simulink model "sm_car_"  (R2026b)
settings: Solver=ode23t  StopTime=100  MaxStep=0.4  AbsTol=1e-3  EnableMultiTasking=on
PreLoadFcn:
  | % Due to usability issue in Repeating Sequence block
  | warning('off','Simulink:Masking:Invalid');
  | 
  | % Eliminate unnecessary warnings in inactive variants
  | % Warnings generated only if you click through inactive variant
  | warning('off','MATLAB:nonExistentField');
  | warning('off','Simulink:Parameters:BlkParamUndefined');
PostLoadFcn:
  | set_param([bdroot '/Vehicle'],'popup_trailer','Off')
  | warning('off','sm:sli:setup:compile:LocalSolverNotSupported')
  | %sm_car_config_maneuver(bdroot,'WOT Braking');
  | sm_car_config_vehicle(bdroot,'false');
  | sm_car_config_logging(bdroot);
InitFcn:
  | sm_car_config_camera;
  | Vehicle = sm_car_vehcfg_checkConfig(Vehicle);
  | sm_car_check_tire_model(bdroot);
StartFcn:
  | tic;
StopFcn:
  | Elapsed_Sim_Time = toc;
  | % disp(['Elapsed Sim Time = ' num2str(Elapsed_Sim_Time)]);
undefined symbols (not defined in the file or in its folder): acc_theta, accel_ramp_rate, Axle1D, AxleIn, Camera, Control, Driver, Init, Maneuver, Pedal, Scene, ShaftL1, ShaftL2, ShaftR1, ShaftR2, Visual, X, xy_data_car_side, Y, Z
libraries: sm_lib x290, fl_lib x171, nesl_utility x144, simulink x60, simulink_extras x14, sdl_lib x14, SimscapeFluids_lib x7, Damper_Element x4, Tire_1x2x x4, ee_lib x3, Scene_Utilities x3, sharedTrackingLibrary x2
(part 8 of 22)

== system sm_car_/Vehicle/Vehicle/Powertrain ==
  CtrlD : Inport
  CtrlP : Inport  Port=2
  VehB : Inport  Port=3
  Driveline : Subsystem  Tag=PublishSubsystem  Variant=on  VariantControlMode=label  VariantControl=Shaft  LabelModeActiveChoice=L2_R2  mask(Variants for Driveline){Driveline=Powertrain.Driveline, VariantLabel=Powertrain.Driveline.class.Value}
      mask prompts: Driveline "Driveline Parameters"; VariantLabel "Variant Label"
      mask help: Select option and provide parameters for driveline. Option is chosen by string provided in Variant Label. The parameters for the selected option are contained in Driveline data structure.
      mask init:
      | curblk = gcb;
      | 
      | % Set variant for this block 
      | set_param(curblk,'LabelModeActiveChoice',VariantLabel);
      settings: AttributesFormatString=%<ActiveVariant>
      mask Help: web('sm_car_doc_driveline.html');
  Power : Subsystem  Variant=on  VariantControlMode=label  VariantControl=Variant1  LabelModeActiveChoice=Electric_L2_R2  mask(Variants for Power){Power=Powertrain.Power, VariantLabel=Powertrain.Power.class.Value}
      mask prompts: Power "Power Parameters"; VariantLabel "Variant Label"
      mask help: Select option and provide parameters for power system (energy storage and actuator). Option is chosen by string provided in Variant Label. The parameters for the selected option are contained in Power data structure.
      mask init:
      | curblk = gcb;
      | 
      | % Set variant for this block 
      | set_param(curblk,'LabelModeActiveChoice',VariantLabel);
      settings: AttributesFormatString=%<ActiveVariant>
  FA : PMIOPort  Side=Left
  Ref : PMIOPort  Port=2  Side=Right
  RA : PMIOPort  Port=3  Side=Right
  R1 : PMIOPort  Port=4  Side=Right
  L1 : PMIOPort  Port=5  Side=Left
  L2 : PMIOPort  Port=6  Side=Left
  R2 : PMIOPort  Port=7  Side=Right
  OutD : Outport  VectorParamsAs1DForOutWhenUnconnected=off
  OutP : Outport  Port=2  VectorParamsAs1DForOutWhenUnconnected=off
  wires:
  Driveline/1(OutD) -> OutD/1
  CtrlD/1 -> Driveline/1(CtrlBus)
  Power/1(OutP) -> OutP/1
  CtrlP/1 -> Power/1(CtrlBus)
  VehB/1 -> Power/2(VehBus)
  connections:
  Driveline/LConn1 -- FA/RConn1
  Ref/RConn1 -- Power/RConn1
  Driveline/RConn1 -- RA/RConn1
  Driveline/LConn4 -- Power/LConn1
  Driveline/LConn2 -- L1/RConn1
  Driveline/RConn2 -- R1/RConn1
  Driveline/RConn3 -- R2/RConn1
  Driveline/LConn3 -- L2/RConn1

== system sm_car_/Vehicle/Vehicle Constraint/No Constraint ==
  F : PMIOPort  Side=Right
  B : PMIOPort  Port=2  Side=Left

== system sm_car_/Vehicle/Vehicle Constraint/No Yaw ==
  Cartesian Joint : sm_lib/Joints/Cartesian Joint  JointMode=Normal  CompositeWrenchDir=FollowerOnBase  CompositeWrenchFrame=BaseFrame  SenseConstraintForce=off  SenseConstraintTorque=off  SenseTotalForce=off  SenseTotalTorque=off  PxPositionTargetSpecify=off  PxPositionTargetPriority=High  PxPositionTargetValue=0  PxPositionTargetValueUnits=m  PxVelocityTargetSpecify=off  PxVelocityTargetPriority=High  PxVelocityTargetValue=0  PxVelocityTargetValueUnits=m/s  PxEquilibriumPosition=0  PxEquilibriumPositionUnits=m  PxSpringStiffness=0  PxSpringStiffnessUnits=N/m  PxDampingCoefficient=0  PxDampingCoefficientUnits=N/(m/s)  PxLowerLimitSpecify=off  PxLowerLimitBound=-1  PxLowerLimitBoundUnits=m  PxLowerLimitStiffness=1e6  PxLowerLimitStiffnessUnits=N/m  PxLowerLimitDamping=1e3  PxLowerLimitDampingUnits=N/(m/s)  PxLowerLimitTransitionRegionWidth=1e-4  PxLowerLimitTransitionRegionWidthUnits=m  PxUpperLimitSpecify=off  PxUpperLimitBound=1  PxUpperLimitBoundUnits=m  PxUpperLimitStiffness=1e6  PxUpperLimitStiffnessUnits=N/m  PxUpperLimitDamping=1e3  PxUpperLimitDampingUnits=N/(m/s)  PxUpperLimitTransitionRegionWidth=1e-4  PxUpperLimitTransitionRegionWidthUnits=m  PxTorqueActuationMode=NoTorque  PxMotionActuationMode=ComputedMotion  PxSensePosition=off  PxSenseVelocity=off  PxSenseAcceleration=off  PxSenseTorqueForce=off  PxSenseLowerLimitTorqueForce=off  PxSenseUpperLimitTorqueForce=off  PyPositionTargetSpecify=off  PyPositionTargetPriority=High  PyPositionTargetValue=0  PyPositionTargetValueUnits=m  PyVelocityTargetSpecify=off  PyVelocityTargetPriority=High  PyVelocityTargetValue=0  PyVelocityTargetValueUnits=m/s  PyEquilibriumPosition=0  PyEquilibriumPositionUnits=m  PySpringStiffness=0  PySpringStiffnessUnits=N/m  PyDampingCoefficient=0  PyDampingCoefficientUnits=N/(m/s)  PyLowerLimitSpecify=off  PyLowerLimitBound=-1  PyLowerLimitBoundUnits=m  PyLowerLimitStiffness=1e6  PyLowerLimitStiffnessUnits=N/m  PyLowerLimitDamping=1e3  PyLowerLimitDampingUnits=N/(m/s)  PyLowerLimitTransitionRegionWidth=1e-4  PyLowerLimitTransitionRegionWidthUnits=m  PyUpperLimitSpecify=off  PyUpperLimitBound=1  PyUpperLimitBoundUnits=m  PyUpperLimitStiffness=1e6  PyUpperLimitStiffnessUnits=N/m  PyUpperLimitDamping=1e3  PyUpperLimitDampingUnits=N/(m/s)  PyUpperLimitTransitionRegionWidth=1e-4  PyUpperLimitTransitionRegionWidthUnits=m  PyTorqueActuationMode=NoTorque  PyMotionActuationMode=ComputedMotion  PySensePosition=off  PySenseVelocity=off  PySenseAcceleration=off  PySenseTorqueForce=off  PySenseLowerLimitTorqueForce=off  PySenseUpperLimitTorqueForce=off  PzPositionTargetSpecify=off  PzPositionTargetPriority=High  PzPositionTargetValue=0  PzPositionTargetValueUnits=m  PzVelocityTargetSpecify=off  PzVelocityTargetPriority=High  PzVelocityTargetValue=0  PzVelocityTargetValueUnits=m/s  PzEquilibriumPosition=0  PzEquilibriumPositionUnits=m  PzSpringStiffness=0  PzSpringStiffnessUnits=N/m  PzDampingCoefficient=0  PzDampingCoefficientUnits=N/(m/s)  PzLowerLimitSpecify=off  PzLowerLimitBound=-1  PzLowerLimitBoundUnits=m  PzLowerLimitStiffness=1e6  PzLowerLimitStiffnessUnits=N/m  PzLowerLimitDamping=1e3  PzLowerLimitDampingUnits=N/(m/s)  PzLowerLimitTransitionRegionWidth=1e-4  PzLowerLimitTransitionRegionWidthUnits=m  PzUpperLimitSpecify=off  PzUpperLimitBound=1  PzUpperLimitBoundUnits=m  PzUpperLimitStiffness=1e6  PzUpperLimitStiffnessUnits=N/m  PzUpperLimitDamping=1e3  PzUpperLimitDampingUnits=N/(m/s)  PzUpperLimitTransitionRegionWidth=1e-4  PzUpperLimitTransitionRegionWidthUnits=m  PzTorqueActuationMode=NoTorque  PzMotionActuationMode=ComputedMotion  PzSensePosition=off  PzSenseVelocity=off  PzSenseAcceleration=off  PzSenseTorqueForce=off  PzSenseLowerLimitTorqueForce=off  PzSenseUpperLimitTorqueForce=off
  Universal Joint : sm_lib/Joints/Universal Joint  JointMode=Normal  CompositeWrenchDir=FollowerOnBase  CompositeWrenchFrame=BaseFrame  SenseConstraintForce=off  SenseConstraintTorque=off  SenseTotalForce=off  SenseTotalTorque=off  RxPositionTargetSpecify=off  RxPositionTargetPriority=High  RxPositionTargetValue=0  RxPositionTargetValueUnits=deg  RxVelocityTargetSpecify=off  RxVelocityTargetPriority=High  RxVelocityTargetValue=0  RxVelocityTargetValueUnits=deg/s  RxEquilibriumPosition=0  RxEquilibriumPositionUnits=deg  RxSpringStiffness=0  RxSpringStiffnessUnits=N*m/deg  RxDampingCoefficient=0  RxDampingCoefficientUnits=N*m/(deg/s)  RxLowerLimitSpecify=off  RxLowerLimitBound=-90  RxLowerLimitBoundUnits=deg  RxLowerLimitStiffness=1e4  RxLowerLimitStiffnessUnits=N*m/deg  RxLowerLimitDamping=10  RxLowerLimitDampingUnits=N*m/(deg/s)  RxLowerLimitTransitionRegionWidth=0.1  RxLowerLimitTransitionRegionWidthUnits=deg  RxUpperLimitSpecify=off  RxUpperLimitBound=90  RxUpperLimitBoundUnits=deg  RxUpperLimitStiffness=1e4  RxUpperLimitStiffnessUnits=N*m/deg  RxUpperLimitDamping=10  RxUpperLimitDampingUnits=N*m/(deg/s)  RxUpperLimitTransitionRegionWidth=0.1  RxUpperLimitTransitionRegionWidthUnits=deg  RxTorqueActuationMode=NoTorque  RxMotionActuationMode=ComputedMotion  RxSensePosition=off  RxSenseVelocity=off  RxSenseAcceleration=off  RxSenseTorqueForce=off  RxSenseLowerLimitTorqueForce=off  RxSenseUpperLimitTorqueForce=off  RyPositionTargetSpecify=off  RyPositionTargetPriority=High  RyPositionTargetValue=0  RyPositionTargetValueUnits=deg  RyVelocityTargetSpecify=off  RyVelocityTargetPriority=High  RyVelocityTargetValue=0  RyVelocityTargetValueUnits=deg/s  RyEquilibriumPosition=0  RyEquilibriumPositionUnits=deg  RySpringStiffness=0  RySpringStiffnessUnits=N*m/deg  RyDampingCoefficient=0  RyDampingCoefficientUnits=N*m/(deg/s)  RyLowerLimitSpecify=off  RyLowerLimitBound=-90  RyLowerLimitBoundUnits=deg  RyLowerLimitStiffness=1e4  RyLowerLimitStiffnessUnits=N*m/deg  RyLowerLimitDamping=10  RyLowerLimitDampingUnits=N*m/(deg/s)  RyLowerLimitTransitionRegionWidth=0.1  RyLowerLimitTransitionRegionWidthUnits=deg  RyUpperLimitSpecify=off  RyUpperLimitBound=90  RyUpperLimitBoundUnits=deg  RyUpperLimitStiffness=1e4  RyUpperLimitStiffnessUnits=N*m/deg  RyUpperLimitDamping=10  RyUpperLimitDampingUnits=N*m/(deg/s)  RyUpperLimitTransitionRegionWidth=0.1  RyUpperLimitTransitionRegionWidthUnits=deg  RyTorqueActuationMode=NoTorque  RyMotionActuationMode=ComputedMotion  RySensePosition=off  RySenseVelocity=off  RySenseAcceleration=off  RySenseTorqueForce=off  RySenseLowerLimitTorqueForce=off  RySenseUpperLimitTorqueForce=off
  F : PMIOPort  Side=Right
  B : PMIOPort  Port=2  Side=Left
  connections:
  Cartesian Joint/LConn1 -- B/RConn1
  Cartesian Joint/RConn1 -- Universal Joint/LConn1
  Universal Joint/RConn1 -- F/RConn1

== system sm_car_/Visualization/Unreal/Animation Off ==
  xyz : Inport
  rpy : Inport  Port=2
  ws : Inport  Port=3
  aCamber : Inport  Port=4
  aSteerWheel : Inport  Port=5
  Terminator{,1..4} (5 alike) : Terminator
  wires:
  rpy/1 -> Terminator1/1
  aSteerWheel/1 -> Terminator4/1
  aCamber/1 -> Terminator3/1
  xyz/1 -> Terminator/1
  ws/1 -> Terminator2/1

== system sm_car_/World/Mechanism Configuration/Constant Gravity ==
  MechanismConfiguration : sm_lib/Utilities/Mechanism Configuration  UniformGravity=Constant  GravityVector=GravityVector  GravityVectorUnits=m/s^2  LinearizationDelta=0.001  JointModeTransitionNonlinearIterations=2
  C : PMIOPort  Side=Right
  connections:
  MechanismConfiguration/RConn1 -- C/RConn1

== system sm_car_/World/Mechanism Configuration/Variable GravityXY ==
  Constant : Constant  Value=acc_theta
  Constant1 : Constant  Value=GravityVector(3)
  MechanismConfiguration : sm_lib/Utilities/Mechanism Configuration  UniformGravity=TimeVarying  GravityVector=[0 0 -9.80665]  GravityVectorUnits=m/s^2  LinearizationDelta=0.001  JointModeTransitionNonlinearIterations=2
  Mux : Mux  Inputs=3
  Product : Product
  Product1 : Product
  Ramp1 : simulink/Sources/Ramp  slope=accel_ramp_rate  start=2  InitialOutput=0
  Scope : Scope
      settings: ActiveDisplayYMinimum=-1.12718  ActiveDisplayYMaximum=10.14459
  Simulink-PS Converter : nesl_utility/Simulink-PS Converter  PhysicalDomain=network_engine_domain  SubClassName=ps_input  LeftPortType=input  RightPortType=output  PseudoPeriodic=off  Frequencies=[]  NoiseDistribution=none  NoiseParameters=[]  Unit=m/s^2  AffineConversion=off  FilteringAndDerivatives=provide  SimscapeFilterOrder=1  InputFilterTimeConstant=0.001  UdotUserProvided=0
  Sin : Trigonometry
  Sin1 : Trigonometry  Operator=cos
  C : PMIOPort  Side=Right
  wires:
  Product/1 -> Mux/2
  Constant/1 -> Sin1/1, Sin/1
  Sin1/1 -> Product1/1
  Mux/1 -> Simulink-PS Converter/1
  Sin/1 -> Product/1
  Constant1/1 -> Mux/3
  Product1/1 -> Mux/1
  Ramp1/1 -> Scope/1, Product1/2, Product/2  "accel_xy"
  connections:
  MechanismConfiguration/RConn1 -- C/RConn1
  MechanismConfiguration/LConn1 -- Simulink-PS Converter/RConn1

== system sm_car_/World/Scene/CRG Hockenheim ==
  Finish Line : Subsystem  mask{post_h=geometry.finish_line.post.height, post_r=geometry.finish_line.post.radius, line_w=geometry.finish_line.post.separation, post_clr=geometry.finish_line.post.clr, post_opc=geometry.finish_line.post.opc, offset_xyz=geometry.finish_line.offset.xyz, offset_yaw=geometry.finish_line.offset.yaw, offset_pitch=geometry.finish_line.offset.pitch, offset_roll=geometry.finish_line.offset.roll}
      mask prompts: post_h "Post Height (m)"; post_r "Post Radius (m)"; line_w "Post Separation (m)"; post_clr "Post Color [R G B] (0-1)"; post_opc "Post Opacity (0-1)"; offset_xyz "Line Offset [x y z] (m)"; offset_yaw "Line Orientation yaw (rad)"; offset_pitch "Line Orientation pitch (rad)"; offset_roll "Line Orientation roll (rad)"
  Ground : Ground
  STL Geometry Centerline : Subsystem  mask{stl_file=geometry.centerline.filename, stl_units=geometry.centerline.fileunits, stl_clr=geometry.centerline.clr, stl_opc=geometry.centerline.opc, stl_x=geometry.centerline.x, stl_y=geometry.centerline.y, stl_z=geometry.centerline.z, stl_yaw=geometry.centerline.yaw, stl_pitch=geometry.centerline.pitch, stl_roll=geometry.centerline.roll}
      mask prompts: stl_file "CAD File"; stl_units "Units"; stl_clr "Color [R G B]"; stl_opc "Opacity (0-1)"; stl_x "Offset x (m)"; stl_y "Offset y (m)"; stl_z "Offset z (m)"; stl_yaw "Offset yaw (rad)"; stl_pitch "Offset pitch (rad)"; stl_roll "Offset roll (rad)"
      mask init:
      | set_param([gcb '/Geometry'],'ExtGeomFileName',stl_file);
      | set_param([gcb '/Geometry'],'ExtGeomFileUnits',stl_units);
  STL Geometry Road : Subsystem  mask{stl_file=geometry.filename, stl_units=geometry.fileunits, stl_clr=geometry.clr, stl_opc=geometry.opc, stl_x=geometry.x, stl_y=geometry.y, stl_z=geometry.z, stl_yaw=geometry.yaw, stl_pitch=geometry.pitch, stl_roll=geometry.roll}
      mask prompts: stl_file "CAD File"; stl_units "Units"; stl_clr "Color [R G B]"; stl_opc "Opacity (0-1)"; stl_x "Offset x (m)"; stl_y "Offset y (m)"; stl_z "Offset z (m)"; stl_yaw "Offset yaw (rad)"; stl_pitch "Offset pitch (rad)"; stl_roll "Offset roll (rad)"
      mask init:
      | set_param([gcb '/Geometry'],'ExtGeomFileName',stl_file);
      | set_param([gcb '/Geometry'],'ExtGeomFileUnits',stl_units);
  W : PMIOPort  Side=Left
  Obs : Outport  VectorParamsAs1DForOutWhenUnconnected=off
  wires:
  Ground/1 -> Obs/1
  connections:
  STL Geometry Centerline/RConn1 -- Finish Line/LConn1 -- W/RConn1 -- STL Geometry Road/RConn1

== system sm_car_/World/Scene/CRG Hockenheim F ==
  Finish Line : Subsystem  mask{post_h=geometry.finish_line.post.height, post_r=geometry.finish_line.post.radius, line_w=geometry.finish_line.post.separation, post_clr=geometry.finish_line.post.clr, post_opc=geometry.finish_line.post.opc, offset_xyz=geometry.finish_line.offset.xyz, offset_yaw=geometry.finish_line.offset.yaw, offset_pitch=geometry.finish_line.offset.pitch, offset_roll=geometry.finish_line.offset.roll}
      mask prompts: post_h "Post Height (m)"; post_r "Post Radius (m)"; line_w "Post Separation (m)"; post_clr "Post Color [R G B] (0-1)"; post_opc "Post Opacity (0-1)"; offset_xyz "Line Offset [x y z] (m)"; offset_yaw "Line Orientation yaw (rad)"; offset_pitch "Line Orientation pitch (rad)"; offset_roll "Line Orientation roll (rad)"
  Ground : Ground
  STL Geometry Centerline : Subsystem  mask{stl_file=geometry.centerline.filename, stl_units=geometry.centerline.fileunits, stl_clr=geometry.centerline.clr, stl_opc=geometry.centerline.opc, stl_x=geometry.centerline.x, stl_y=geometry.centerline.y, stl_z=geometry.centerline.z, stl_yaw=geometry.centerline.yaw, stl_pitch=geometry.centerline.pitch, stl_roll=geometry.centerline.roll}
      mask prompts: stl_file "CAD File"; stl_units "Units"; stl_clr "Color [R G B]"; stl_opc "Opacity (0-1)"; stl_x "Offset x (m)"; stl_y "Offset y (m)"; stl_z "Offset z (m)"; stl_yaw "Offset yaw (rad)"; stl_pitch "Offset pitch (rad)"; stl_roll "Offset roll (rad)"
      mask init:
      | set_param([gcb '/Geometry'],'ExtGeomFileName',stl_file);
      | set_param([gcb '/Geometry'],'ExtGeomFileUnits',stl_units);
  STL Geometry Road : Subsystem  mask{stl_file=geometry.filename, stl_units=geometry.fileunits, stl_clr=geometry.clr, stl_opc=geometry.opc, stl_x=geometry.x, stl_y=geometry.y, stl_z=geometry.z, stl_yaw=geometry.yaw, stl_pitch=geometry.pitch, stl_roll=geometry.roll}
      mask prompts: stl_file "CAD File"; stl_units "Units"; stl_clr "Color [R G B]"; stl_opc "Opacity (0-1)"; stl_x "Offset x (m)"; stl_y "Offset y (m)"; stl_z "Offset z (m)"; stl_yaw "Offset yaw (rad)"; stl_pitch "Offset pitch (rad)"; stl_roll "Offset roll (rad)"
      mask init:
      | set_param([gcb '/Geometry'],'ExtGeomFileName',stl_file);
      | set_param([gcb '/Geometry'],'ExtGeomFileUnits',stl_units);
  W : PMIOPort  Side=Left
  Obs : Outport  VectorParamsAs1DForOutWhenUnconnected=off
  wires:
  Ground/1 -> Obs/1
  connections:
  STL Geometry Centerline/RConn1 -- Finish Line/LConn1 -- W/RConn1 -- STL Geometry Road/RConn1

== system sm_car_/World/Scene/Double Lane Change ==
  Cones Double Lane Change : Scene_Utilities/Cones Double Lane Change  lane_width=cones.lane_width  lane_separation=cones.lane_lateral_offset  start_lane_a=cones.lane_a_offset  A1_to_A5=cones.lane_a_length  A_to_B_x=cones.gap_a_to_b  B1_to_B5=cones.lane_b_length  B_to_C_x=cones.gap_b_to_c  C1_to_C5=cones.lane_c_length  height=cones.height  baseThickness=cones.base_thickness  baseWidth=cones.base_width  coneBaseDiameter=cones.bottom_diameter  coneTopDiameter=cones.top_diameter  reflectiveStripHeight=cones.strip_height  coneColor=cones.clr  reflectiveStripColor=cones.strip_clr
  Dashes : Scene_Utilities/Dashes  dash_pitch=dashes.pitch  num_dashes=dashes.num  dash_l=dashes.l  dash_h=dashes.h  dash_w=dashes.w  thickness_base=dashes.base_h  dash_clr=dashes.clr  dash_opc=dashes.opc
  Ground : Ground
  Road : Scene_Utilities/Patch Rectangle  gp_l=road.l  gp_w=road.w  gp_h=road.h  gp_clr=road.clr  gp_opc=road.opc
  Transform Cones : sm_lib/Frames and Transforms/Rigid Transform  RotationMethod=None  FollAlignAxisA=+X  BaseAlignAxisA=+Y  FollAlignAxisB=+Y  BaseAlignAxisB=+Z  RotationStandardAxis=+Z  RotationAngle=0.0  RotationAngleUnits=deg  RotationArbitraryAxis=[0 0 1]  RotationSequenceAxes=FollowerAxes  RotationSequence=XYX  RotationSequenceAngles=[0 0 0]  RotationSequenceAnglesUnits=deg  RotationMatrix=[1 0 0; 0 1 0; 0 0 1]  Quaternion=[1 0 0 0]  TranslationMethod=StandardAxis  TranslationCartesianOffset=[0 0 0]  TranslationCartesianOffsetUnits=m  TranslationStandardAxis=-X  TranslationStandardOffset=road.l/2  TranslationStandardOffsetUnits=m  TranslationROffset=0  TranslationROffsetUnits=m  TranslationThetaOffset=0  TranslationThetaOffsetUnits=deg  TranslationZOffset=0  TranslationZOffsetUnits=m
  Transform Road : sm_lib/Frames and Transforms/Rigid Transform  RotationMethod=RotationSequence  FollAlignAxisA=+X  BaseAlignAxisA=+Y  FollAlignAxisB=+Y  BaseAlignAxisB=+Z  RotationStandardAxis=+Z  RotationAngle=0.0  RotationAngleUnits=deg  RotationArbitraryAxis=[0 0 1]  RotationSequenceAxes=BaseAxes  RotationSequence=ZYX  RotationSequenceAngles=[road.yaw road.pitch road.roll]  RotationSequenceAnglesUnits=rad  RotationMatrix=[1 0 0; 0 1 0; 0 0 1]  Quaternion=[1 0 0 0]  TranslationMethod=Cartesian  TranslationCartesianOffset=[road.x road.y road.z]  TranslationCartesianOffsetUnits=m  TranslationStandardAxis=+Z  TranslationStandardOffset=0  TranslationStandardOffsetUnits=m  TranslationROffset=0  TranslationROffsetUnits=m  TranslationThetaOffset=0  TranslationThetaOffsetUnits=deg  TranslationZOffset=0  TranslationZOffsetUnits=m
  W : PMIOPort  Side=Left
  Obs : Outport  VectorParamsAs1DForOutWhenUnconnected=off
  wires:
  Ground/1 -> Obs/1
  connections:
  W/RConn1 -- Transform Road/LConn1
  Dashes/LConn1 -- Road/RConn1 -- Transform Cones/LConn1 -- Transform Road/RConn1
  Cones Double Lane Change/LConn1 -- Transform Cones/RConn1

== system sm_car_/World/Scene/Plane Grid ==
  Grid : Subsystem  mask{grid_x=plane.l, grid_y=plane.w, grid_z=plane.h, grid_line_width=grid.line_width, grid_num_sq_x=grid.num_sqrs_x, grid_num_sq_y=grid.num_sqrs_y, grid_clr=grid.clr, grid_opc=grid.opc}
      mask prompts: grid_x "Length (m) (Global x)"; grid_y "Width (m) (Global y)"; grid_z "Depth (m) (Global z)"; grid_line_width "Line width (m)"; grid_num_sq_x "Number of squares in x"; grid_num_sq_y "Number of squares in y"; grid_clr "Color [RGB]"; grid_opc "Opacity (0-1)"
      mask init:
      | % Derived parameters - for two perpendicular grids with num_sq-by-1 holes
      | % **Note, not num_sq_x by num_sq_y holes - better render speed with
      | % separate meshes for x and y.
      | 
      | hole_lx = (grid_x-(grid_line_width*(grid_num_sq_x+1)))/grid_num_sq_x;
      | hole_wx = (grid_y-(grid_line_width*(1+1)))/1;
      | 
      | hole_ly = (grid_y-(grid_line_width*(grid_num_sq_y+1)))/grid_num_sq_y;
      | hole_wy = (grid_x-(grid_line_width*(1+1)))/1;
  Ground : Ground
  Ground Plane : Subsystem  mask{gp_l=plane.l, gp_w=plane.w, gp_h=plane.h, gp_clr=plane.clr, gp_opc=plane.opc}
      mask prompts: gp_l "Length (m) (Global  x)"; gp_w "Width (m) (Global  y)"; gp_h "Depth (m) (Global z)"; gp_clr "Color [R G B]"; gp_opc "Opacity (0-1)"
  Transform Plane : sm_lib/Frames and Transforms/Rigid Transform  RotationMethod=None  FollAlignAxisA=+X  BaseAlignAxisA=+Y  FollAlignAxisB=+Y  BaseAlignAxisB=+Z  RotationStandardAxis=+Z  RotationAngle=0.0  RotationAngleUnits=deg  RotationArbitraryAxis=[0 0 1]  RotationSequenceAxes=FollowerAxes  RotationSequence=XYX  RotationSequenceAngles=[0 0 0]  RotationSequenceAnglesUnits=deg  RotationMatrix=[1 0 0; 0 1 0; 0 0 1]  Quaternion=[1 0 0 0]  TranslationMethod=Cartesian  TranslationCartesianOffset=[plane.x plane.y plane.z]  TranslationCartesianOffsetUnits=m  TranslationStandardAxis=+Z  TranslationStandardOffset=0  TranslationStandardOffsetUnits=m  TranslationROffset=0  TranslationROffsetUnits=m  TranslationThetaOffset=0  TranslationThetaOffsetUnits=deg  TranslationZOffset=0  TranslationZOffsetUnits=m
  W : PMIOPort  Side=Left
  Obs : Outport  VectorParamsAs1DForOutWhenUnconnected=off
  wires:
  Ground/1 -> Obs/1
  connections:
  Ground Plane/RConn1 -- Transform Plane/RConn1 -- Grid/LConn1
  Transform Plane/LConn1 -- W/RConn1

== system sm_car_/World/Scene/Skidpad ==
  Circle Inner L : Subsystem  mask{circ_d=circ_in.d, circ_a1=-180, circ_a2=180, circ_w=circ_in.w, circ_h=circ_in.h, circ_clr=circ_in.clr, circ_opc=circ_in.opc}
      mask prompts: circ_d "Circle Diameter (m)"; circ_a1 "Start Angle (deg)"; circ_a2 "Finish Angle (deg)"; circ_w "Stripe Width (m)"; circ_h "Stripe Height (m)"; circ_clr "Color [RGB]"; circ_opc "Opacity (0-1)"
      mask init:
      | xy_data_circ = Extr_Data_Ring(...
      |     circ_d/2+circ_w/2,circ_d/2-circ_w/2,circ_a1, circ_a2);
  Circle Inner R : Subsystem  mask{circ_d=circ_in.d, circ_a1=-180, circ_a2=180, circ_w=circ_in.w, circ_h=circ_in.h, circ_clr=circ_in.clr, circ_opc=circ_in.opc}
      mask prompts: circ_d "Circle Diameter (m)"; circ_a1 "Start Angle (deg)"; circ_a2 "Finish Angle (deg)"; circ_w "Stripe Width (m)"; circ_h "Stripe Height (m)"; circ_clr "Color [RGB]"; circ_opc "Opacity (0-1)"
      mask init:
      | xy_data_circ = Extr_Data_Ring(...
      |     circ_d/2+circ_w/2,circ_d/2-circ_w/2,circ_a1, circ_a2);
  Circle Outer L : Subsystem  mask{circ_d=circ_out.d, circ_a1=circ_out.ang1, circ_a2=circ_out.ang2, circ_w=circ_out.w, circ_h=circ_out.h, circ_clr=circ_out.clr, circ_opc=circ_out.opc}
      mask prompts: circ_d "Circle Diameter (m)"; circ_a1 "Start Angle (deg)"; circ_a2 "Finish Angle (deg)"; circ_w "Stripe Width (m)"; circ_h "Stripe Height (m)"; circ_clr "Color [RGB]"; circ_opc "Opacity (0-1)"
      mask init:
      | xy_data_circ = Extr_Data_Ring(...
      |     circ_d/2+circ_w/2,circ_d/2-circ_w/2,circ_a1, circ_a2);
  Circle Outer R : Subsystem  mask{circ_d=circ_out.d, circ_a1=circ_out.ang1, circ_a2=circ_out.ang2, circ_w=circ_out.w, circ_h=circ_out.h, circ_clr=circ_out.clr, circ_opc=circ_out.opc}
      mask prompts: circ_d "Circle Diameter (m)"; circ_a1 "Start Angle (deg)"; circ_a2 "Finish Angle (deg)"; circ_w "Stripe Width (m)"; circ_h "Stripe Height (m)"; circ_clr "Color [RGB]"; circ_opc "Opacity (0-1)"
      mask init:
      | xy_data_circ = Extr_Data_Ring(...
      |     circ_d/2+circ_w/2,circ_d/2-circ_w/2,circ_a1, circ_a2);
  Ground : Ground
  Ground Plane : Subsystem  mask{gp_l=plane.l, gp_w=plane.w, gp_h=plane.h, gp_clr=plane.clr, gp_opc=plane.opc}
      mask prompts: gp_l "Length (m) (Global  x)"; gp_w "Width (m) (Global  y)"; gp_h "Depth (m) (Global z)"; gp_clr "Color [R G B]"; gp_opc "Opacity (0-1)"
  Transform Circle L : sm_lib/Frames and Transforms/Rigid Transform  RotationMethod=None  FollAlignAxisA=+X  BaseAlignAxisA=+Y  FollAlignAxisB=+Y  BaseAlignAxisB=+Z  RotationStandardAxis=+Z  RotationAngle=0.0  RotationAngleUnits=deg  RotationArbitraryAxis=[0 0 1]  RotationSequenceAxes=FollowerAxes  RotationSequence=XYX  RotationSequenceAngles=[0 0 0]  RotationSequenceAnglesUnits=deg  RotationMatrix=[1 0 0; 0 1 0; 0 0 1]  Quaternion=[1 0 0 0]  TranslationMethod=Cartesian  TranslationCartesianOffset=[0 circ_in.sep/2 0]  TranslationCartesianOffsetUnits=m  TranslationStandardAxis=+Z  TranslationStandardOffset=0  TranslationStandardOffsetUnits=m  TranslationROffset=0  TranslationROffsetUnits=m  TranslationThetaOffset=0  TranslationThetaOffsetUnits=deg  TranslationZOffset=0  TranslationZOffsetUnits=m
  Transform Circle R : sm_lib/Frames and Transforms/Rigid Transform  RotationMethod=None  FollAlignAxisA=+X  BaseAlignAxisA=+Y  FollAlignAxisB=+Y  BaseAlignAxisB=+Z  RotationStandardAxis=+Z  RotationAngle=0.0  RotationAngleUnits=deg  RotationArbitraryAxis=[0 0 1]  RotationSequenceAxes=FollowerAxes  RotationSequence=XYX  RotationSequenceAngles=[0 0 0]  RotationSequenceAnglesUnits=deg  RotationMatrix=[1 0 0; 0 1 0; 0 0 1]  Quaternion=[1 0 0 0]  TranslationMethod=Cartesian  TranslationCartesianOffset=[0 -circ_in.sep/2 0]  TranslationCartesianOffsetUnits=m  TranslationStandardAxis=+Z  TranslationStandardOffset=0  TranslationStandardOffsetUnits=m  TranslationROffset=0  TranslationROffsetUnits=m  TranslationThetaOffset=0  TranslationThetaOffsetUnits=deg  TranslationZOffset=0  TranslationZOffsetUnits=m
  Transform Orient OuterL : sm_lib/Frames and Transforms/Rigid Transform  RotationMethod=StandardAxis  FollAlignAxisA=+X  BaseAlignAxisA=+Y  FollAlignAxisB=+Y  BaseAlignAxisB=+Z  RotationStandardAxis=+Z  RotationAngle=90  RotationAngleUnits=deg  RotationArbitraryAxis=[0 0 1]  RotationSequenceAxes=FollowerAxes  RotationSequence=XYX  RotationSequenceAngles=[0 0 0]  RotationSequenceAnglesUnits=deg  RotationMatrix=[1 0 0; 0 1 0; 0 0 1]  Quaternion=[1 0 0 0]  TranslationMethod=None  TranslationCartesianOffset=[0 0 0]  TranslationCartesianOffsetUnits=m  TranslationStandardAxis=+Z  TranslationStandardOffset=0  TranslationStandardOffsetUnits=m  TranslationROffset=0  TranslationROffsetUnits=m  TranslationThetaOffset=0  TranslationThetaOffsetUnits=deg  TranslationZOffset=0  TranslationZOffsetUnits=m
  Transform Orient OuterR : sm_lib/Frames and Transforms/Rigid Transform  RotationMethod=StandardAxis  FollAlignAxisA=+X  BaseAlignAxisA=+Y  FollAlignAxisB=+Y  BaseAlignAxisB=+Z  RotationStandardAxis=+Z  RotationAngle=-90  RotationAngleUnits=deg  RotationArbitraryAxis=[0 0 1]  RotationSequenceAxes=FollowerAxes  RotationSequence=XYX  RotationSequenceAngles=[0 0 0]  RotationSequenceAnglesUnits=deg  RotationMatrix=[1 0 0; 0 1 0; 0 0 1]  Quaternion=[1 0 0 0]  TranslationMethod=None  TranslationCartesianOffset=[0 0 0]  TranslationCartesianOffsetUnits=m  TranslationStandardAxis=+Z  TranslationStandardOffset=0  TranslationStandardOffsetUnits=m  TranslationROffset=0  TranslationROffsetUnits=m  TranslationThetaOffset=0  TranslationThetaOffsetUnits=deg  TranslationZOffset=0  TranslationZOffsetUnits=m
  Transform Plane : sm_lib/Frames and Transforms/Rigid Transform  RotationMethod=None  FollAlignAxisA=+X  BaseAlignAxisA=+Y  FollAlignAxisB=+Y  BaseAlignAxisB=+Z  RotationStandardAxis=+Z  RotationAngle=0.0  RotationAngleUnits=deg  RotationArbitraryAxis=[0 0 1]  RotationSequenceAxes=FollowerAxes  RotationSequence=XYX  RotationSequenceAngles=[0 0 0]  RotationSequenceAnglesUnits=deg  RotationMatrix=[1 0 0; 0 1 0; 0 0 1]  Quaternion=[1 0 0 0]  TranslationMethod=Cartesian  TranslationCartesianOffset=[plane.x plane.y plane.z]  TranslationCartesianOffsetUnits=m  TranslationStandardAxis=+Z  TranslationStandardOffset=0  TranslationStandardOffsetUnits=m  TranslationROffset=0  TranslationROffsetUnits=m  TranslationThetaOffset=0  TranslationThetaOffsetUnits=deg  TranslationZOffset=0  TranslationZOffsetUnits=m
  W : PMIOPort  Side=Left
  Obs : Outport  VectorParamsAs1DForOutWhenUnconnected=off
  wires:
  Ground/1 -> Obs/1
  connections:
  Circle Outer L/RConn1 -- Transform Orient OuterL/RConn1
  Circle Outer R/RConn1 -- Transform Orient OuterR/RConn1
  Circle Inner R/RConn1 -- Transform Circle R/RConn1 -- Transform Orient OuterR/LConn1
  Transform Plane/RConn1 -- Ground Plane/RConn1
  Transform Circle L/LConn1 -- W/RConn1 -- Transform Plane/LConn1 -- Transform Circle R/LConn1
  Circle Inner L/RConn1 -- Transform Circle L/RConn1 -- Transform Orient OuterL/LConn1

== system sm_car_/Controller/Default/Brake Control/Pedal ==
  rBrakePedal : Inport
  VehBus : Inport  Port=2
  Apply{,1..3} (4 alike) : Constant  Value=[0 1]
  Bus Creator : BusCreator  Inputs=1
  Bus Creator1 : BusCreator  Inputs=4
  Terminator : Terminator
  Terminator1 : Terminator
  Brakes : Outport  VectorParamsAs1DForOutWhenUnconnected=off
  wires:
  rBrakePedal/1 -> Terminator1/1
  Apply3/1 -> Bus Creator1/4  "R2"
  Apply2/1 -> Bus Creator1/3  "L2"
  Apply1/1 -> Bus Creator1/2  "R1"
  Apply/1 -> Bus Creator1/1  "L1"
  Bus Creator1/1 -> Bus Creator/1  "Valves"
  VehBus/1 -> Terminator/1
  Bus Creator/1 -> Brakes/1  "Brakes"

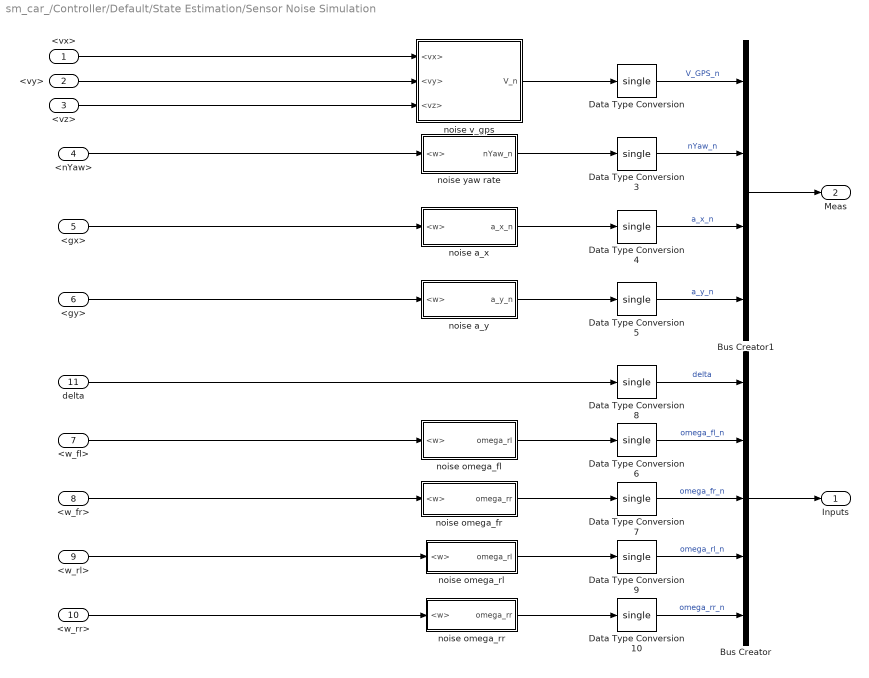
== system sm_car_/Controller/Default/State Estimation/Sensor Noise Simulation ==
  <vx> : Inport
  <vy> : Inport  Port=2
  <vz> : Inport  Port=3
  <nYaw> : Inport  Port=4
  <gx> : Inport  Port=5
  <gy> : Inport  Port=6
  <w_fl> : Inport  Port=7
  <w_fr> : Inport  Port=8
  <w_rl> : Inport  Port=9
  <w_rr> : Inport  Port=10
  delta : Inport  Port=11
  Bus Creator : BusCreator  Inputs=5
  Bus Creator1 : BusCreator  Inputs=4
  Data Type Conversion{,3..10} (9 alike) : DataTypeConversion  OutDataTypeStr=single  SaturateOnIntegerOverflow=off  RndMeth=Floor
  noise a_x : Subsystem
  noise a_y : Subsystem
  noise omega_fl : Subsystem
  noise omega_fr : Subsystem
  noise omega_rl : Subsystem
  noise omega_rr : Subsystem
  noise v_gps : Subsystem
  noise yaw rate : Subsystem
  Inputs : Outport
  Meas : Outport  Port=2
  wires:
  delta/1 -> Data Type Conversion8/1
  <w_fl>/1 -> noise omega_fl/1(<w>)
  <nYaw>/1 -> noise yaw rate/1(<w>)
  <w_fr>/1 -> noise omega_fr/1(<w>)
  <gx>/1 -> noise a_x/1(<w>)
  noise a_x/1(a_x_n) -> Data Type Conversion4/1
  <vx>/1 -> noise v_gps/1(<vx>)
  noise omega_fl/1(omega_rl) -> Data Type Conversion6/1
  noise a_y/1(a_y_n) -> Data Type Conversion5/1
  Bus Creator/1 -> Inputs/1
  noise omega_rl/1(omega_rl) -> Data Type Conversion9/1
  noise yaw rate/1(nYaw_n) -> Data Type Conversion3/1
  <w_rl>/1 -> noise omega_rl/1(<w>)
  <gy>/1 -> noise a_y/1(<w>)
  noise omega_rr/1(omega_rr) -> Data Type Conversion10/1
  <w_rr>/1 -> noise omega_rr/1(<w>)
  noise omega_fr/1(omega_rr) -> Data Type Conversion7/1
  Bus Creator1/1 -> Meas/1
  Data Type Conversion/1 -> Bus Creator1/1  "V_GPS_n"
  Data Type Conversion3/1 -> Bus Creator1/2  "nYaw_n"
  Data Type Conversion4/1 -> Bus Creator1/3  "a_x_n"
  Data Type Conversion5/1 -> Bus Creator1/4  "a_y_n"
  Data Type Conversion6/1 -> Bus Creator/2  "omega_fl_n"
  Data Type Conversion7/1 -> Bus Creator/3  "omega_fr_n"
  Data Type Conversion8/1 -> Bus Creator/1  "delta"
  Data Type Conversion9/1 -> Bus Creator/4  "omega_rl_n"
  Data Type Conversion10/1 -> Bus Creator/5  "omega_rr_n"
  noise v_gps/1(V_n) -> Data Type Conversion/1
  <vy>/1 -> noise v_gps/2(<vy>)
  <vz>/1 -> noise v_gps/3(<vz>)

== system sm_car_/Controller/Default/State Estimation/UKF ==
  StateTransitionFcnInputs : Inport  PortDimensions=5
  y1 : Inport  Port=2
  Compare To Constant : simulink/Logic and Bit Operations/Compare To Constant  relop=<=  const=0.5  OutDataTypeStr=boolean
  Constant : Constant  Value=0  OutDataTypeStr=single  SampleTime=0.003
  Constant1 : Constant  Value=0  OutDataTypeStr=single
  Delay : Delay  DelayLength=1  SampleTime=0.003
  Demux : Demux  Outputs=5
  MATLAB Function : MATLAB Function  TreatAsAtomicUnit=on
  Mux : Mux  Inputs=5
  Switch : Switch  Criteria=u2 ~= 0  SaturateOnIntegerOverflow=off  InputSameDT=off
  Unscented Kalman Filter : sharedTrackingLibrary/Unscented Kalman Filter  StateTransitionFcn=prediction_model  HasAdditiveProcessNoise=Additive  ProcessNoise=diag([1e-5, 8e-6, 1e-6, 5e-5, 1e-4])  HasTimeVaryingProcessNoise=on  HasStateTransitionFcnExtraArgument=1  InitialState=[0.4; 0; 0; 0; 0]  InitialStateCovariance=diag([0.04, 0.04, 1e-3, 0.1, 0.1])  Alpha=0.1  Beta=2  Kappa=0  MeasurementFcn1=measurement_model  HasMeasurementEnablePort1=off  HasAdditiveMeasurementNoise1=Additive  MeasurementNoise1=[9e-4, 7.29e-7, 1.22e-4, 1.22e-4]  HasTimeVaryingMeasurementNoise1=off  HasMeasurementFcnExtraArgument1=1  HasMeasurementWrapping1=on  MeasurementFcn2=myMeasurementFcn  HasMeasurementEnablePort2=off  HasAdditiveMeasurementNoise2=Additive  MeasurementNoise2=1  HasTimeVaryingMeasurementNoise2=off  HasMeasurementFcnExtraArgument2=0  HasMeasurementWrapping2=off  MeasurementFcn3=myMeasurementFcn  HasMeasurementEnablePort3=off  HasAdditiveMeasurementNoise3=Additive  MeasurementNoise3=1  HasTimeVaryingMeasurementNoise3=off  HasMeasurementFcnExtraArgument3=0  HasMeasurementWrapping3=off  MeasurementFcn4=myMeasurementFcn  HasMeasurementEnablePort4=off  HasAdditiveMeasurementNoise4=Additive  MeasurementNoise4=1  HasTimeVaryingMeasurementNoise4=off  HasMeasurementFcnExtraArgument4=0  HasMeasurementWrapping4=off  MeasurementFcn5=myMeasurementFcn  HasMeasurementEnablePort5=off  HasAdditiveMeasurementNoise5=Additive  MeasurementNoise5=1  HasTimeVaryingMeasurementNoise5=off  HasMeasurementFcnExtraArgument5=0  HasMeasurementWrapping5=off  EnableMultirate=off  StateTransitionFcnSampleTime=1  MeasurementFcn1SampleTime=1  MeasurementFcn2SampleTime=1  MeasurementFcn3SampleTime=1  MeasurementFcn4SampleTime=1  MeasurementFcn5SampleTime=1  UseCurrentEstimator=on  OutputStateCovariance=off  DataType=single  SampleTime=0.003  NumberOfMeasurements=1
      settings: LibrarySourceBlock=cstblocks/State Estimation/Unscented Kalman Filter
  xhat : Outport
  wires:
  y1/1 -> Unscented Kalman Filter/3
  StateTransitionFcnInputs/1 -> Unscented Kalman Filter/2
  Constant/1 -> Unscented Kalman Filter/4
  Unscented Kalman Filter/1 -> Delay/1, Demux/1
  MATLAB Function/1(Q) -> Unscented Kalman Filter/1
  Delay/1 -> MATLAB Function/1(xhat)
  Compare To Constant/1 -> Switch/2
  Constant1/1 -> Switch/1
  Demux/1 -> Mux/1, Compare To Constant/1
  Demux/2 -> Switch/3
  Switch/1 -> Mux/2
  Demux/3 -> Mux/3
  Demux/4 -> Mux/4
  Demux/5 -> Mux/5
  Mux/1 -> xhat/1

== system sm_car_/Controller/FeedF_Ctrl/Brake Control/Pedal ==
  rBrakePedal : Inport
  VehBus : Inport  Port=2
  Apply{,1..3} (4 alike) : Constant  Value=[0 1]
  Bus Creator : BusCreator  Inputs=1
  Bus Creator1 : BusCreator  Inputs=4
  Terminator : Terminator
  Terminator1 : Terminator
  Brakes : Outport  VectorParamsAs1DForOutWhenUnconnected=off
  wires:
  Bus Creator/1 -> Brakes/1  "Brakes"
  VehBus/1 -> Terminator/1
  Bus Creator1/1 -> Bus Creator/1  "Valves"
  Apply/1 -> Bus Creator1/1  "L1"
  Apply1/1 -> Bus Creator1/2  "R1"
  Apply2/1 -> Bus Creator1/3  "L2"
  Apply3/1 -> Bus Creator1/4  "R2"
  rBrakePedal/1 -> Terminator1/1

== system sm_car_/Controller/NoIMU/Brake Control/Pedal ==
  rBrakePedal : Inport
  VehBus : Inport  Port=2
  Apply{,1..3} (4 alike) : Constant  Value=[0 1]
  Bus Creator : BusCreator  Inputs=1
  Bus Creator1 : BusCreator  Inputs=4
  Terminator : Terminator
  Terminator1 : Terminator
  Brakes : Outport  VectorParamsAs1DForOutWhenUnconnected=off
  wires:
  Bus Creator/1 -> Brakes/1  "Brakes"
  VehBus/1 -> Terminator/1
  Bus Creator1/1 -> Bus Creator/1  "Valves"
  Apply/1 -> Bus Creator1/1  "L1"
  Apply1/1 -> Bus Creator1/2  "R1"
  Apply2/1 -> Bus Creator1/3  "L2"
  Apply3/1 -> Bus Creator1/4  "R2"
  rBrakePedal/1 -> Terminator1/1

== system sm_car_/Controller/NoIMU/Power Control/Current-Torque ==
  note: modify to accomade all voltage ranges
      | only 220V now
  note: current - torque
  V : Inport
  Il : Inport  Port=2
  Ir : Inport  Port=3
  Add : Sum
  Km : Gain  Gain=Km
  Km1 : Gain  Gain=Km
  Terminator : Terminator
  Out1 : Outport
  wires:
  Il/1 -> Km1/1
  Km1/1 -> Add/1
  V/1 -> Terminator/1
  Ir/1 -> Km/1
  Add/1 -> Out1/1
  Km/1 -> Add/2

== system sm_car_/Controller/NoIMU/Power Control/Slip Control ==
  VehBus : Inport
  Bus Selector : BusSelector  OutputSignals=Power.MotorL2.w,Power.MotorL2.i,Power.MotorR2.w,Power.MotorR2.i
  Constant : Constant
  Constant1 : Constant  Value=0
  I no load : Constant  Value=I0
  Product : Product
  Product1 : Product
  Relational Operator : RelationalOperator  OutDataTypeStr=boolean  RndMeth=Simplest  InputSameDT=off
  Relational Operator1 : RelationalOperator  Operator=<=  OutDataTypeStr=boolean  RndMeth=Simplest  InputSameDT=off
  Relational Operator2 : RelationalOperator  OutDataTypeStr=boolean  RndMeth=Simplest  InputSameDT=off
  Relational Operator3 : RelationalOperator  Operator=<=  OutDataTypeStr=boolean  RndMeth=Simplest  InputSameDT=off
  Switch : Switch  Criteria=u2 > Threshold  SaturateOnIntegerOverflow=off  InputSameDT=off
  Switch1 : Switch  Criteria=u2 > Threshold  SaturateOnIntegerOverflow=off  InputSameDT=off
  w no load : Constant  Value=w0
  Out1 : Outport
  Out2 : Outport  Port=2
  wires:
  VehBus/1 -> Bus Selector/1
  Bus Selector/1 -> Relational Operator/1  "<w>"
  Product/1 -> Switch/2
  Relational Operator/1 -> Product/1
  Relational Operator1/1 -> Product/2
  Relational Operator2/1 -> Product1/1
  Relational Operator3/1 -> Product1/2
  Product1/1 -> Switch1/2
  Constant1/1 -> Switch/3, Switch1/3
  Constant/1 -> Switch1/1, Switch/1
  Bus Selector/2 -> Relational Operator1/1  "<i>"
  Bus Selector/3 -> Relational Operator2/1  "<w>"
  Bus Selector/4 -> Relational Operator3/1  "<i>"
  I no load/1 -> Relational Operator1/2, Relational Operator3/2
  w no load/1 -> Relational Operator/2, Relational Operator2/2
  Switch/1 -> Out1/1
  Switch1/1 -> Out2/1

== system sm_car_/Controller/Slip_Ctrl/Brake Control/Pedal ==
  rBrakePedal : Inport
  VehBus : Inport  Port=2
  Apply{,1..3} (4 alike) : Constant  Value=[0 1]
  Bus Creator : BusCreator  Inputs=1
  Bus Creator1 : BusCreator  Inputs=4
  Terminator : Terminator
  Terminator1 : Terminator
  Brakes : Outport  VectorParamsAs1DForOutWhenUnconnected=off
  wires:
  Bus Creator/1 -> Brakes/1  "Brakes"
  VehBus/1 -> Terminator/1
  Bus Creator1/1 -> Bus Creator/1  "Valves"
  Apply/1 -> Bus Creator1/1  "L1"
  Apply1/1 -> Bus Creator1/2  "R1"
  Apply2/1 -> Bus Creator1/3  "L2"
  Apply3/1 -> Bus Creator1/4  "R2"
  rBrakePedal/1 -> Terminator1/1

== system sm_car_/Controller/Slip_Ctrl_V2/Brake Control/Pedal ==
  rBrakePedal : Inport
  VehBus : Inport  Port=2
  Apply{,1..3} (4 alike) : Constant  Value=[0 1]
  Bus Creator : BusCreator  Inputs=1
  Bus Creator1 : BusCreator  Inputs=4
  Terminator : Terminator
  Terminator1 : Terminator
  Brakes : Outport  VectorParamsAs1DForOutWhenUnconnected=off
  wires:
  rBrakePedal/1 -> Terminator1/1
  Apply3/1 -> Bus Creator1/4  "R2"
  Apply2/1 -> Bus Creator1/3  "L2"
  Apply1/1 -> Bus Creator1/2  "R1"
  Apply/1 -> Bus Creator1/1  "L1"
  Bus Creator1/1 -> Bus Creator/1  "Valves"
  VehBus/1 -> Terminator/1
  Bus Creator/1 -> Brakes/1  "Brakes"

== system sm_car_/Controller/TrqVec 4Motor/Brake Control/ABS ==
  rBrakePedal : Inport
  In Bus Element1 : Inport  Port=2  PortName=VehBus  Element=Chassis
  In Bus Element2 : Inport  Port=2  PortName=VehBus  Element=Chassis.Body.CG
  Bus Creator1 : BusCreator  Inputs=4
  Bus Creator2 : BusCreator  Inputs=1
  Bus Selector : BusSelector  OutputSignals=L1
  Bus Selector1 : BusSelector  OutputSignals=R1
  Bus Selector2 : BusSelector  OutputSignals=L2
  Bus Selector3 : BusSelector  OutputSignals=R2
  Calculate Slip : Subsystem
  Sensor : Subsystem
  Terminator : Terminator
  Valve Control L1 : Subsystem
  Valve Control L2 : Subsystem
  Valve Control R1 : Subsystem
  Valve Control R2 : Subsystem
  Vehicle Speed : Subsystem
  Brakes : Outport  VectorParamsAs1DForOutWhenUnconnected=off
  wires:
  rBrakePedal/1 -> Terminator/1
  Vehicle Speed/1(vSpdEst) -> Valve Control R2/2(vSpdEst), Valve Control L2/2(vSpdEst), Valve Control R1/2(vSpdEst), Valve Control L1/2(vSpdEst), Calculate Slip/2(VehSpdEst)
  Sensor/1(GroundSpd) -> Vehicle Speed/1(Sensors), Calculate Slip/1(WhlSpd)
  Bus Creator1/1 -> Bus Creator2/1  "Valves"
  Bus Selector2/1 -> Valve Control L2/1(Slip)  "<L2>"
  Valve Control R1/1(Valve) -> Bus Creator1/2  "R1"
  Valve Control R2/1(Valve) -> Bus Creator1/4  "R2"
  Valve Control L2/1(Valve) -> Bus Creator1/3  "L2"
  Bus Selector3/1 -> Valve Control R2/1(Slip)  "<R2>"
  Bus Selector/1 -> Valve Control L1/1(Slip)  "<L1>"
  Calculate Slip/1(Slip) -> Bus Selector3/1, Bus Selector2/1, Bus Selector1/1, Bus Selector/1
  Valve Control L1/1(Valve) -> Bus Creator1/1  "L1"
  Bus Selector1/1 -> Valve Control R1/1(Slip)  "<R1>"
  Bus Creator2/1 -> Brakes/1  "Brakes"
  In Bus Element1/1 -> Sensor/2(WhlSpd)
  In Bus Element2/1 -> Sensor/1(Body)

== system sm_car_/Controller/TrqVec 4Motor/Brake Control/Pedal ==
  rBrakePedal : Inport
  VehBus : Inport  Port=2
  Apply{,1..3} (4 alike) : Constant  Value=[0 1]
  Bus Creator : BusCreator  Inputs=1
  Bus Creator1 : BusCreator  Inputs=4
  Terminator : Terminator
  Terminator1 : Terminator
  Brakes : Outport  VectorParamsAs1DForOutWhenUnconnected=off
  wires:
  rBrakePedal/1 -> Terminator1/1
  Apply3/1 -> Bus Creator1/4  "R2"
  Apply2/1 -> Bus Creator1/3  "L2"
  Apply1/1 -> Bus Creator1/2  "R1"
  Apply/1 -> Bus Creator1/1  "L1"
  Bus Creator1/1 -> Bus Creator/1  "Valves"
  VehBus/1 -> Terminator/1
  Bus Creator/1 -> Brakes/1  "Brakes"

== system sm_car_/Controller/TrqVec 4Motor/Brake Control/Pressure ==
  rBrakePedal : Inport
  VehBus : Inport  Port=2
  Bus Creator : BusCreator  Inputs=4
  Gain : Gain  Gain=Vehicle.Brakes.Front.Caliper.pMax.Value
  Gain1 : Gain  Gain=Vehicle.Brakes.Front.Caliper.pMax.Value
  Gain2 : Gain  Gain=Vehicle.Brakes.Rear.Caliper.pMax.Value
  Gain3 : Gain  Gain=Vehicle.Brakes.Rear.Caliper.pMax.Value
  Terminator : Terminator
  Brakes : Outport  VectorParamsAs1DForOutWhenUnconnected=off
  wires:
  rBrakePedal/1 -> Gain/1, Gain1/1, Gain3/1, Gain2/1
  VehBus/1 -> Terminator/1
  Bus Creator/1 -> Brakes/1  "Brakes"
  Gain/1 -> Bus Creator/1  "pBrakeL1"
  Gain1/1 -> Bus Creator/2  "pBrakeR1"
  Gain2/1 -> Bus Creator/3  "pBrakeL2"
  Gain3/1 -> Bus Creator/4  "pBrakeR2"

== system sm_car_/Controller/TrqVec 4Motor/Power_TqVec/Torque Vectoring ==
  trqA2 : Inport
  vx : Inport  Port=2
  aSteerWheel : Inport  Port=3
  wL2 : Inport  Port=4
  wR2 : Inport  Port=5
  nYaw : Inport  Port=6
  rBrake : Inport  Port=7
  Accel Torque Request : Subsystem
  Calculate Torque Split : MATLAB Function  TreatAsAtomicUnit=on
  Compare To Constant1 : simulink/Logic and Bit Operations/Compare To Constant  relop=<  const=.01  OutDataTypeStr=boolean
  Data Type Conversion : DataTypeConversion  SaturateOnIntegerOverflow=off  RndMeth=Floor
  Enable : Subsystem
  Gain1 : Gain  Gain=0.5
  Gain5 : Gain
  Gain6 : Gain
  Max Delta Torque : Constant  Value=max_torque_delta
  PID Controller : slpidlib/PID Controller  Controller=PID  Form=Parallel  TimeDomain=Continuous-time  UseExternalTs=off  SampleTime=-1  IntegratorMethod=Forward Euler  FilterMethod=Forward Euler  ControllerParametersSource=internal  P=P  I=I  UseKiTs=off  D=0  UseExternalDerivativeSource=off  N=1  UseFilter=on  TunerSelectOption=Transfer Function Based (PID Tuner App)  InitialConditionSource=internal  InitialConditionForIntegrator=0  InitialConditionForFilter=0  DifferentiatorICPrevScaledInput=0  ExternalReset=either  TrackingMode=off  Kt=1  LimitOutput=off  SatLimitsSource=internal  UpperSaturationLimit=inf  LowerSaturationLimit=-inf  LinearizeAsGain=on  AntiWindupMode=back-calculation  Kb=1  LimitIntegrator=off  UpperIntegratorSaturationLimit=inf  LowerIntegratorSaturationLimit=-inf  POutMin=[]  POutMax=[]  IOutMin=[]  IOutMax=[]  DOutMin=[]  DOutMax=[]  NOutMin=[]  NOutMax=[]  SumOutMin=[]  SumOutMax=[]  SaturationOutMin=[]  SaturationOutMax=[]  PParamMin=[]  PParamMax=[]  IParamMin=[]  IParamMax=[]  DParamMin=[]  DParamMax=[]  NParamMin=[]  NParamMax=[]  KbParamMin=[]  KbParamMax=[]  KtParamMin=[]  KtParamMax=[]  KbOutMin=[]  KbOutMax=[]  KtOutMin=[]  KtOutMax=[]  IntegratorOutMin=[]  IntegratorOutMax=[]  FilterOutMin=[]  FilterOutMax=[]  SumI1OutMin=[]  SumI1OutMax=[]  SumI2OutMin=[]  SumI2OutMax=[]  SumI3OutMin=[]  SumI3OutMax=[]  SumI4OutMin=[]  SumI4OutMax=[]  SumDOutMin=[]  SumDOutMax=[]  DifferentiatorOutMin=[]  DifferentiatorOutMax=[]  FilterDiffOutCoefMin=[]  FilterDiffOutCoefMax=[]  ReciprocalOutMin=[]  ReciprocalOutMax=[]  SumDenOutMin=[]  SumDenOutMax=[]  SumNumOutMin=[]  SumNumOutMax=[]  DivideOutMin=[]  DivideOutMax=[]  UdiffTsProdOutMin=[]  UdiffTsProdOutMax=[]  NTsProdOutMin=[]  NTsProdOutMax=[]  UintegralTsProdOutMin=[]  UintegralTsProdOutMax=[]  UngainTsProdOutMin=[]  UngainTsProdOutMax=[]  ClampingZeroOutDataTypeStr=Inherit: Inherit via back propagation  ClampingZeroOutMin=[]  ClampingZeroOutMax=[]  FilterDenConstantOutDataTypeStr=Inherit: Inherit via back propagation  FilterDenConstantOutMin=[]  FilterDenConstantOutMax=[]  PCopyOutDataTypeStr=Inherit: Inherit via back propagation  PCopyOutMin=[]  PCopyOutMax=[]  NCopyOutDataTypeStr=Inherit: Inherit via back propagation  NCopyOutMin=[]  NCopyOutMax=[]  IntegratorContinuousStateAttributes=''  IntegratorStateMustResolveToSignalObject=off  IntegratorRTWStateStorageClass=Auto  FilterContinuousStateAttributes=''  FilterStateMustResolveToSignalObject=off  FilterRTWStateStorageClass=Auto  ParallelPVariant=InternalParameters  IdealPVariant=Disabled  IVariant=InternalParameters  DVariant=InternalParameters  IntegratorVariant=Continuous  SatVariant=Disabled  AWVariant=Passthrough  PCopyVariant=Disabled  TRVariant=Disabled  FdbkBlocksVariant=Forward  IdealPFdbkVariant=Disabled  SatFdbkVariant=Disabled  DerivativeFilterVariant=ContFilter  NVariant=InternalParameters  NCopyVariant=Disabled  FilterICVariant=InternalICsFilter  IntegratorICVariant=InternalICs  ExternalResetVariant=ExternalReset  TRSumVariant=Passthrough  SumFdbkVariant=Disabled  SumVariant=Sum_PID  TsampFilterVariant=InternalTs  TsampNgainVariant=Passthrough  TsampIntegralVariant=Disabled_SignalSpec  ExternalSaturationOutDataTypeStr=Inherit: Same as second input  DerivativeSourceVariant=ErrorSignal  PreIntVariant=InternalPreInt
  Transfer Fcn : TransferFcn  Denominator=[0.5 1]
  Transfer Fcn1 : TransferFcn  Denominator=[.001 1]
  Transfer Fcn2 : TransferFcn  Denominator=[.001 1]
  Vehicle Slip Angle Error : Subsystem
  trqL2 : Outport  VectorParamsAs1DForOutWhenUnconnected=off
  trqR2 : Outport  Port=2  VectorParamsAs1DForOutWhenUnconnected=off
  wires:
  Compare To Constant1/1 -> Data Type Conversion/1
  Data Type Conversion/1 -> Transfer Fcn/1
  Max Delta Torque/1 -> Calculate Torque Split/2(max_delta_trq)
  nYaw/1 -> Vehicle Slip Angle Error/3(nYaw)
  Enable/1(Enable) -> Calculate Torque Split/1(enable), PID Controller/2  "Enable"
  Gain1/1 -> Calculate Torque Split/4(tq_l), Calculate Torque Split/5(tq_r)
  rBrake/1 -> Compare To Constant1/1
  Gain6/1 -> trqR2/1
  Vehicle Slip Angle Error/1(Error) -> PID Controller/1
  Calculate Torque Split/1(tq_l_out) -> Gain5/1
  Transfer Fcn/1 -> Calculate Torque Split/7(brk)
  Transfer Fcn2/1 -> Accel Torque Request/2(MotSpdR2)
  trqA2/1 -> Gain1/1
  Calculate Torque Split/2(tq_r_out) -> Gain6/1
  wR2/1 -> Transfer Fcn2/1
  PID Controller/1 -> Calculate Torque Split/6(tq_tv)
  Gain5/1 -> trqL2/1
  aSteerWheel/1 -> Enable/2(aSteerWheel), Vehicle Slip Angle Error/2(aSteerWheel)
  vx/1 -> Enable/1(vx), Vehicle Slip Angle Error/1(vx)
  Accel Torque Request/1(TrqMax) -> Calculate Torque Split/3(max_tq)
  Transfer Fcn1/1 -> Accel Torque Request/1(MotSpdL2)
  wL2/1 -> Transfer Fcn1/1
